simulink model "Twin_Builder"  (R2026a)
settings: Solver=VariableStepAuto  StopTime=simTime  FixedStep=Ts/60  RelTol=1e-2
values from neighbouring files (symbols this model uses):
  ac = log(9)/tr    [Run_Twin.m]
  as = 0.08 * ac    [Run_Twin.m]
  ath = 0.25 * as    [Run_Twin.m]
  B = 0.00001    (= 1e-05)    [Run_Twin.m]
  BEMFD_FEA_PerHz = InterpFEA_Data_ForSimulink(FEA_Data.BackEMFD_perHz, IS_FEA, IEA_FEA, IS_Interp, IEA_Interp)    [Run_Twin.m]
  BEMFQ_FEA_PerHz = InterpFEA_Data_ForSimulink(FEA_Data.BackEMFQ_perHz, IS_FEA, IEA_FEA, IS_Interp, IEA_Interp)    [Run_Twin.m]
  CondLoss_Inv = zeros([length(IS_Interp), size(FEA_Data.ConductionLoss, [2 3] ) ])    [Run_Twin.m]
  CopperLoss_FEA = InterpFEA_Data_ForSimulink(FEA_Data.CopperLosses, IS_FEA, IEA_FEA, IS_Interp, IEA_Interp)    [Run_Twin.m]
  DriveMethod = 1    [Run_Twin.m]
  EnvTorque_FW = interp1(Speed_full, Env_full, Speed_Vec, 'pchip', 'extrap')    [Run_Twin.m]
  f_sw = 10e3    (= 10000)    [Run_Twin.m]
  FEA_Data = LoadData.(FieldData{1})    [Run_Twin.m]
  FILTER_COEFF = 0.23    [Run_Twin.m]
  FluxD_FEA = InterpFEA_Data_ForSimulink(FEA_Data.FluxD, IS_FEA, IEA_FEA, IS_Interp, IEA_Interp)    [Run_Twin.m]
  FluxQ_FEA = InterpFEA_Data_ForSimulink(FEA_Data.FluxQ, IS_FEA, IEA_FEA, IS_Interp, IEA_Interp)    [Run_Twin.m]
  FrictLoss_FEA = squeeze( FEA_Data.FrictLosses(1,1,:) )    [Run_Twin.m]
  GateLoss_Inv = zeros([length(IS_Interp), size(FEA_Data.ConductionLoss, [2 3] ) ])    [Run_Twin.m]
  IDcore_FEA = InterpFEA_Data_ForSimulink(FEA_Data.IDc, IS_FEA, IEA_FEA, IS_Interp, IEA_Interp)    [Run_Twin.m]
  IEA_FEA = IEA_Interp    [Run_Twin.m]
  IQcore_FEA = InterpFEA_Data_ForSimulink(FEA_Data.IQc, IS_FEA, IEA_FEA, IS_Interp, IEA_Interp)    [Run_Twin.m]
  IronLoss_FEA = InterpFEA_Data_ForSimulink(FEA_Data.IronLosses,   IS_FEA, IEA_FEA, IS_Interp, IEA_Interp)    [Run_Twin.m]
  Is_Amp = 40    [Run_Twin.m]
  IS_FEA = IS_Interp    [Run_Twin.m]
  J = FEA_Data.Jinertia    [Run_Twin.m]
  J_Control = FEA_Data.Jinertia    [Run_Twin.m]
  LD_FEA = InterpFEA_Data_ForSimulink(FEA_Data.LD, IS_FEA, IEA_FEA, IS_Interp, IEA_Interp)    [Run_Twin.m]
  LD_Single = mean(LD_FEA, 'all')    [Run_Twin.m]
  LQ_FEA = InterpFEA_Data_ForSimulink(FEA_Data.LQ, IS_FEA, IEA_FEA, IS_Interp, IEA_Interp)    [Run_Twin.m]
  LQ_Single = mean(LQ_FEA, 'all')    [Run_Twin.m]
  MagnetLoss_FEA = InterpFEA_Data_ForSimulink(FEA_Data.MagnetLosses, IS_FEA, IEA_FEA, IS_Interp, IEA_Interp)    [Run_Twin.m]
  MaxSpeed = max(Speed_Vec)    [Run_Twin.m]
  MaxTe = max(Torque_FEA, [], 'all')    [Run_Twin.m]
  ModStrategy = 1    [Run_Twin.m]
  PMFlux_FEA = interp1(IS_FEA, squeeze( FEA_Data.FluxD(:,IEA_FEA == 90, :) ), IS_Interp, 'pchip' )    [Run_Twin.m]
  PMFlux_Single = mean( PMFlux_FEA, 'all' )    [Run_Twin.m]
  PMT_ID = round( F_ID(PMT_grid, Speed_grid), 2)    [Run_Twin.m]
  PMT_IQ = round( F_IQ(PMT_grid, Speed_grid), 2)    [Run_Twin.m]
  PMT_Vec = linspace(0,   100,   InterpSamples)    [Run_Twin.m]
  PolePair = FEA_Data.Poles / 2    [Run_Twin.m]
  PPR = 1024    [Run_Twin.m]
  ProxiLoss_FEA = InterpFEA_Data_ForSimulink(FEA_Data.ProxiLosses,  IS_FEA, IEA_FEA, IS_Interp, IEA_Interp)    [Run_Twin.m]
  Rcore_FEA = InterpFEA_Data_ForSimulink(FEA_Data.Rcore, IS_FEA, IEA_FEA, IS_Interp, IEA_Interp)    [Run_Twin.m]
  RDC = squeeze( Rseries_FEA(1,1,1) )    [Run_Twin.m]
  RefSpeed = [50, 400, 250, 500, 400]    [Run_Twin.m]
  RefTheta = [50, 0, 140, 300, -50]    [Run_Twin.m]
  Rseries_FEA = InterpFEA_Data_ForSimulink(FEA_Data.Rs,    IS_FEA, IEA_FEA, IS_Interp, IEA_Interp)    [Run_Twin.m]
  ShafthLoad = [10, 25, 3, 8, 10]    [Run_Twin.m]
  simTime = mechThetaTarget / wMechTarget    [Run_Twin.m]
  Speed_FEA = FEA_Data.Speed_vec    [Run_Twin.m]
  Speed_Vec = linspace(min(Speed_full), max(Speed_full), InterpSamples)    [Run_Twin.m]
  speedTarget = 200    [Run_Twin.m]
  SR_FEA = FEA_Data.SynchAngle    [Run_Twin.m]
  SwitchLoss_Inv = zeros([length(IS_Interp), size(FEA_Data.ConductionLoss, [2 3] ) ])    [Run_Twin.m]
  Tdt = 0.3 * 1e-6    (= 3e-07)    [Run_Twin.m]
  Throttle = 45    [Run_Twin.m]
  Times = [0, 0.2, 0.4, 0.6, 0.8] * simTime    [Run_Twin.m]
  Torque_FEA = InterpFEA_Data_ForSimulink(FEA_Data.TorqueFEA, IS_FEA, IEA_FEA, IS_Interp, IEA_Interp)    [Run_Twin.m]
  Ts = 1/f_sw    (= 0.0001)    [Run_Twin.m]
  Ts_Sp = 2 * Ts    (= 0.0002)    [Run_Twin.m]
  Vdc = 56    [Run_Twin.m]
  Vs_pu = 0.98    [Run_Twin.m]
  WindageLoss_FEA = squeeze( FEA_Data.WindLosses(1,1,:) )    [Run_Twin.m]
undefined symbols (not defined in the file or in its folder): DiscIntNeverNeededParam, feNom, mf, OverMod, PMT_Speed, SimData, Tables
libraries: simulink x14, ee_lib x11, simulink_extras x7, eeTransforms x6, fl_lib x6, eeGeneralControl x4, spsMeanLib x2, dspxfrm3 x1
(part 3 of 3)

== matlab function Twin_Builder/Inverter/Create VRef/Determine Common Mode Signal/CommonModeSignal ==
  settings: updateMethod=DISCRETE  sampleTime=Ts
  data: ModStrategy input; CommonMode output; SPWM input; SVPWM input; THIPWM input; THZSPWM input; DPWM1 input; DPWMMAX input; DPWMMIN input
function CommonMode  = fcn(ModStrategy, SPWM, SVPWM, THIPWM, THZSPWM, DPWM1, DPWMMAX, DPWMMIN)

switch ModStrategy
    case 0
        CommonMode = SPWM;
    case 1
        CommonMode = SVPWM;
    case 2
        CommonMode = THIPWM;
    case 3
        CommonMode = THZSPWM;
    case 4
        CommonMode = DPWM1;
    case 5
        CommonMode = DPWMMAX;     
    case 6
        CommonMode = DPWMMIN;     
          
    otherwise
        error('Invalid ModStrategy: must be 0 to 4');
end

== matlab function Twin_Builder/Inverter/Create VRef/Determine Common Mode Signal/MATLAB Function ==
  data: ModStrategy input; OverMod output; OverMod_Ampl input
function OverMod = fcn(ModStrategy, OverMod_Ampl)

if ModStrategy == 0
    OverMod = 1/OverMod_Ampl;
    
else 
    OverMod = 1;

end

== matlab function Twin_Builder/Inverter/Create VRef/Determine Common Mode Signal/DPWMMAX Technique ==
  settings: updateMethod=DISCRETE  sampleTime=Ts
  data: VaRef input; Vcommon output; VbRef input; VcRef input
function Vcommon  = fcn(VaRef, VbRef, VcRef)

% Find the maximum phase reference voltage
Vmax    = max([VaRef, VbRef, VcRef]);

% DPWMMAX common-mode voltage calculation
Vcommon = - (Vmax - 1.0);

== matlab function Twin_Builder/Controller/Control Process/VDQ Reference from Voltage Controller/Determine Control ==
  settings: updateMethod=DISCRETE  sampleTime=Ts
  data: u input; y output
function y  = fcn(u)
y = 1;
if u == 0
  y = 1;
else 
  y = 0;
end


end

== matlab function Twin_Builder/Inverter/Create VRef/Determine Common Mode Signal/DPWMMIN Technique ==
  settings: updateMethod=DISCRETE  sampleTime=Ts
  data: VaRef input; Vcommon output; VbRef input; VcRef input
function Vcommon  = fcn(VaRef, VbRef, VcRef)

% Find the minimum phase reference voltage
Vmin = min([VaRef, VbRef, VcRef]);

% Compute the common mode voltage using DPWMMIN logic
Vcommon = - (Vmin + 1.0);

== matlab function Twin_Builder/Controller/Control Process/IDQ _Reference/Determine Torque Control ==
  settings: updateMethod=DISCRETE  sampleTime=Ts
  data: u input; y output
function y  = fcn(u)
y = 1;
if u == 3 
  y = 1;
else 
  y = 0;
end


end

== matlab function Twin_Builder/PMSM /LUTS/Treat Angles >180 & <1 ==
  settings: updateMethod=CONTINUOUS
  data: u input; y output
function y  = fcn(u)
y =u;
if u>180
  y = 360-u;
end
if u<0
  y = -u;
end

end

== matlab function Twin_Builder/Controller/Update Speed Ref ==
  settings: updateMethod=DISCRETE
  data: ChangeTimes input; Time input; Value output; Values input
function Value = fcn(ChangeTimes, Time, Values)

Value = UpdateSignal(ChangeTimes, Time, Values);

== matlab function Twin_Builder/PMSM /LUTS/QEP /Sample θ ==
  settings: updateMethod=DISCRETE  sampleTime=Ts_Sp
  data: theta input; Ts input; omega output; delta_theta output; FILTER_COEFF input
function [omega, delta_theta] = fcn(theta, Ts, FILTER_COEFF)

[omega, delta_theta] = Speed_From_Theta(theta, Ts, FILTER_COEFF);

== matlab function Twin_Builder/Controller/Control Process/IDQ References from Speed Controller/Update Speed Ref ==
  settings: updateMethod=DISCRETE
  data: TeCommand input; IEA_Command input; IdRef output; Psimag input; Ld input; Lq input; PolePair input; IqRef output
function [IdRef, IqRef] = fcn(TeCommand, IEA_Command, Psimag, Ld, Lq, PolePair)

[IdRef, IqRef] = Current_From_Torque(TeCommand, IEA_Command, Psimag, Ld, Lq, PolePair);

== matlab function Twin_Builder/Controller/Control Process/Speed Reference from Position Controller/Determine Position Control ==
  settings: updateMethod=DISCRETE  sampleTime=Ts
  data: u input; y output
function y  = fcn(u)
y = 1;
if u == 4 
  y = 1;
else 
  y = 0;
end

== matlab function Twin_Builder/Controller/Control Process/Speed Reference from Position Controller/Determine Speed Control ==
  settings: updateMethod=DISCRETE  sampleTime=Ts
  data: u input; y output
function y  = fcn(u)
y = 1;
if u == 2 
  y = 1;
else 
  y = 0;
end

== matlab function Twin_Builder/Controller/Control Process/IDQ _Reference/Determine Speed Control ==
  settings: updateMethod=DISCRETE  sampleTime=Ts
  data: u input; y output
function y  = fcn(u)
y = 1;
if u == 2 || u == 4
  y = 1;
else 
  y = 0;
end


end

== matlab function Twin_Builder/PMSM /Quantize Electrical Theta  ==
  settings: updateMethod=DISCRETE  sampleTime=Ts
  data: theta_w input; PPR input; Theta_mcu output; Count output
function [Theta_mcu, Count] = QuantizeTheta_Caller(theta_w, PPR)
% Emulates encoder counter reading (MCU)
% 1024 PPR, x4 decoding => 4096 counts/rev

[Theta_mcu, Count] = QuantizeTheta(theta_w, PPR);

== matlab function Twin_Builder/Controller/Update Speed Ref1 ==
  settings: updateMethod=DISCRETE
  data: ChangeTimes input; Time input; Value output; Values input
function Value = fcn(ChangeTimes, Time, Values)

Value = UpdateSignal(ChangeTimes, Time, Values);

== matlab function Twin_Builder/PMSM /Update Load1 ==
  settings: updateMethod=DISCRETE
  data: ChangeTimes input; Time input; Value output; Values input
function Value = fcn(ChangeTimes, Time, Values)

Value = UpdateSignal(ChangeTimes, Time, Values);

end

== matlab function Twin_Builder/Controller/Control Process/IDQ _Reference/Determine Current Control ==
  settings: updateMethod=DISCRETE  sampleTime=Ts
  data: u input; y output
function y  = fcn(u)
y = 1;
if u == 1 
  y = 1;
else 
  y = 0;
end

== matlab function Twin_Builder/PMSM /LUTS/Sample Currents ==
  settings: updateMethod=DISCRETE
  data: Signal input; TriSignal input; SampledSignals output
function SampledSignals = fcn(Signal, TriSignal)

SampledSignals = SampleSignals(Signal, TriSignal);

end

== matlab function Twin_Builder/PMSM /LUTS/SimulinkToMatlab/Sample VREF ==
  settings: updateMethod=DISCRETE
  data: Signal input; TriSignal input; SampledSignal output
function SampledSignal = fcn(Signal, TriSignal)

SampledSignal = SampleSignals(Signal, TriSignal);

== matlab function Twin_Builder/Controller/Control Process/VDQ Reference from Current Controller Fundamental/Determine Control ==
  settings: updateMethod=DISCRETE  sampleTime=Ts
  data: u input; y output
function y  = fcn(u)
y = 1;
if u == 1 || u == 2 ||  u == 3 ||  u == 4
  y = 1;
else 
  y = 0;
end

== matlab function Twin_Builder/PMSM /LUTS/QEP /Quantize Electrical Theta  ==
  settings: updateMethod=DISCRETE  sampleTime=Ts
  data: theta_w input; PPR input; Theta_mcu output; Count output
function [Theta_mcu, Count] = QuantizeTheta_Caller(theta_w, PPR)
% Emulates encoder counter reading (MCU)
% 1024 PPR, x4 decoding => 4096 counts/rev

[Theta_mcu, Count] = QuantizeTheta(theta_w, PPR);

== matlab function Twin_Builder/PMSM /LUTS/Fix NaN IDcore ==
  data: u input; y output
function y = fcn(u)

y  = ReplaceNaNInfs(u);

end

== matlab function Twin_Builder/PMSM /LUTS/Fix NaN IQcore ==
  data: u input; y output
function y = fcn(u)

y  = ReplaceNaNInfs(u);

end

== matlab function Twin_Builder/PMSM /LUTS/If Iq <0 Invert Torque ==
  settings: updateMethod=CONTINUOUS  sampleTime=Ts
  data: u input; y output
function y  = fcn(u)

if u < 0
  y = -1;

else 
  y = 1;
end


end

== matlab function Twin_Builder/PMSM /LUTS/Treat Angles >180 & <0 ==
  settings: updateMethod=CONTINUOUS
  data: u input; y output
function y  = fcn(u)
y =u;
if u>180
  y = 360-u;
end
if u<0
  y = -u;
end

end

== matlab function Twin_Builder/Inverter/Create VRef/Sample References ==
  settings: updateMethod=DISCRETE
  data: Signal input; TriSignal input; SampledSignals output
function SampledSignals = fcn(Signal, TriSignal)

SampledSignals = SampleSignals(Signal, TriSignal);
